simulink model "model_PWM_dspic"  (Simulink 7.4)
settings: Solver=FixedStepDiscrete  StartTime=0.0  StopTime=0.08  FixedStep=0.00001  RelTol=1e-3
undefined symbols (not defined in the file or in its folder): DiscIntNeverNeededParam
libraries: dsPICdrivers x7
settings Model: Creator=ELMAY  LastModifiedBy=ELMAY
settings OptimizationCC: OptimizeModelRefInitCode=on  LifeSpan=1
settings HardwareCC: ProdBitPerInt=16  ProdEndianess=LittleEndian  ProdWordSize=16  ProdHWDeviceType=16-bit Generic
settings RTWCC: SystemTargetFile=dspic.tlc  MakeCommand=make_CreateMPLAB  TemplateMakefile=dspic_pic30_gcc.tmf  PostCodeGenCommand=dsPIC_Compile()  Description=Embedded Target for Microchip dsPIC (real-time)  GenerateReport=on  ProcessScript=dspic_make_rtw_hook  IncludeHyperlinkInReport=on  LaunchReport=on
settings CodeAppCC: IgnoreCustomStorageClasses=off
settings STFCustomTargetCC: IncludeMdlTerminateFcn=off  CombineOutputUpdateFcns=on  SuppressErrorStatus=on  ERTCustomFileBanners=on  SupportContinuousTime=off  SupportNonInlinedSFcns=off  SystemTargetFile=dspic.tlc
settings ERTTargetCC: MultiwordLength=2048  ParMdlRefBuildCompliant=off  CompOptLevelCompliant=off  IncludeMdlTerminateFcn=off  SuppressErrorStatus=on  ERTFirstTimeCompliant=off  ModelStepFunctionPrototypeControlCompliant=off  CPPClassGenCompliant=off  ExtModeMexFile=ext_serial_win32_comm  InlinedParameterPlacement=NonHierarchical  ERTSrcFileBannerTemplate=dsPIC_code_template.cgt  ERTHdrFileBannerTemplate=dsPIC_code_template.cgt  ERTDataSrcFileTemplate=dsPIC_code_template.cgt  ERTDataHdrFileTemplate=dsPIC_code_template.cgt  ERTCustomFileTemplate=dsPIC_main.tlc  ConvertIfToSwitch=off
settings CustomProperty: DataType=string  Value=D:\PROGRA~1\MATLAB\R2009b\bin\win32\gmake

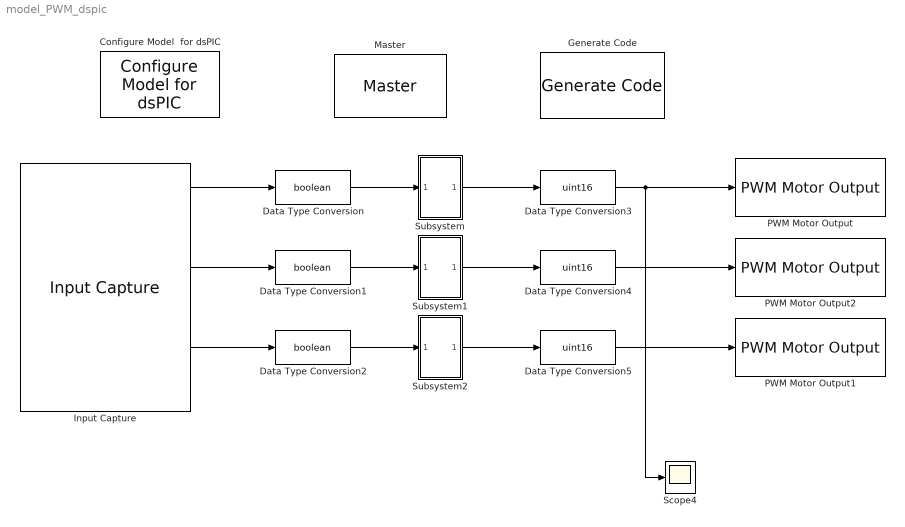
== system model_PWM_dspic ==
  Configure Model  for dsPIC : dsPICdrivers/Simulink Configuration/Configure Model  for dsPIC
  Data Type Conversion : DataTypeConversion  OutDataTypeMode=boolean  OutDataType=sfix(16)  OutScaling=2^0  OutDataTypeStr=boolean
  Data Type Conversion1 : DataTypeConversion  OutDataTypeMode=boolean  OutDataType=sfix(16)  OutScaling=2^0  OutDataTypeStr=boolean
  Data Type Conversion2 : DataTypeConversion  OutDataTypeMode=boolean  OutDataType=sfix(16)  OutScaling=2^0  OutDataTypeStr=boolean
  Data Type Conversion3 : DataTypeConversion  OutDataTypeMode=uint16  OutDataType=sfix(16)  OutScaling=2^0  OutDataTypeStr=uint16
  Data Type Conversion4 : DataTypeConversion  OutDataTypeMode=uint16  OutDataType=sfix(16)  OutScaling=2^0  OutDataTypeStr=uint16
  Data Type Conversion5 : DataTypeConversion  OutDataTypeMode=uint16  OutDataType=sfix(16)  OutScaling=2^0  OutDataTypeStr=uint16
  Generate Code : dsPICdrivers/Simulink Configuration/Generate Code
  Input Capture : dsPICdrivers/Peripheral I//O/Input Capture  Tag=dsPIC_PWM_IC  Priority=5  IntPriority=7  Channel="[ 1 2  7]"  Channel_UP_Down_Periode="[5  5  5]"  MaxChannel="[0.01        0.01        0.01]"  SafeMarge="[10  10  10]"  MaxName=' IC1max , IC2max , IC7max '  Precision="[13.8725      13.8725      13.8725]"  Timer="[2  2  2]"  ChangeDetected="[0  0  0]"  ChangeDetectedPortRef=3  SampleTime=-1  Status=OK
  Master : dsPICdrivers/Master  Tag=dsPIC_MASTER  Priority=1  TimeStepType=Timer1  picType=30f4011  fcy=12e6  Quartz_33f=5e6  PLLActive_33f=off  fcyDesired_33f=0  tmr1="[1  119  1.1842e-014]"  tmr1Info="Time Step : 1e-005  ;   Error : 1.1842e-014%  PR1=119"  tmr2345="[8  0  0  0]"  tmr2345cfg=[-1 -1 -1 -1]  IOautoConf=on  typePort="[ 0  0  0  0  0  0  0  0  0  0  0  0  0  0  0  0  0  0  0  0  6  6  0  0  0  0  0  0  0  0  0  0  0  0  0  0  0  0  0  0  0  0  0  0  0  0  0  0  6  0  0  0  0  0  0  0  0  0  0  0  0  0  0  0  0  0  0  0  0  0  0  0  0  0  0  0  0  0  0  0  0  0  0  0  0  0  0  0  0  0  0  0  0  0  0  0  0  0  0  0  0  0  0  0  0  0  0  0  0  0  0  0 ]"  TRIS="[ 65535  65535  65535  65535  65535  65535  65535 ]"  ADPCFG=48  MasterBusyPort=None  MasterOverloadPort=None  FOSC=HS  ClockSwitchMonitor=Both disabled  TempProtection_33f=TEMP_ON  FPBOR=PBOR_OFF  PWRT=PWRT_OFF  MCLR=MCLR_DIS  ICD=ICS_PGD1  JTAGEN=JTAGEN_OFF  PowerSave=off  OverrideFcy=off  NewFcy=1e6  PR2345="[65535  65535  65535  65535]"
  PWM Motor Output : dsPICdrivers/Peripheral I//O/PWM Motor Output  Tag=dsPIC_PWM_Motor  Priority=5  PWMref=1  PWM12=1  InputEnableChk=off  InputPeriodeChk=off  Channel=[1 ]  TPeriode=0.02  PrescalerValue=16  PeriodeInteger=15000  MaxName='PWM'  Centered=off  HChannelON=off  Info="Nbr Bits : 14.8727  ||  PWM = 30000  ||  Prescaler = 16"  Delay=0  IntPriority=5  nbrPwmChannelPIC=3  Status=OK  DeadTimePrescaleA=0  DeadTimePrescaleB=0  DeadTimeInfo=Dead Time A = 0  DTPWM1a=Prescaler A  DTPWM1i=Prescaler A  DTPWM2a=Prescaler A  DTPWM2i=Prescaler A  DTPWM3a=Prescaler A  DTPWM3i=Prescaler A  DTPWM4a=Prescaler A  DTPWM4i=Prescaler A  DTCON1=0  DTCON2=0
  PWM Motor Output1 : dsPICdrivers/Peripheral I//O/PWM Motor Output  Tag=dsPIC_PWM_Motor  Priority=5  PWMref=1  PWM12=1  InputEnableChk=off  InputPeriodeChk=off  Channel=[3 ]  TPeriode=0.02  PrescalerValue=16  PeriodeInteger=15000  MaxName='PWM'  Centered=off  HChannelON=off  Info="Nbr Bits : 14.8727  ||  PWM = 30000  ||  Prescaler = 16"  Delay=0  IntPriority=5  nbrPwmChannelPIC=3  Status=OK  DeadTimePrescaleA=0  DeadTimePrescaleB=0  DeadTimeInfo=Dead Time A = 0  DTPWM1a=Prescaler A  DTPWM1i=Prescaler A  DTPWM2a=Prescaler A  DTPWM2i=Prescaler A  DTPWM3a=Prescaler A  DTPWM3i=Prescaler A  DTPWM4a=Prescaler A  DTPWM4i=Prescaler A  DTCON1=0  DTCON2=0
  PWM Motor Output2 : dsPICdrivers/Peripheral I//O/PWM Motor Output  Tag=dsPIC_PWM_Motor  Priority=5  PWMref=1  PWM12=1  InputEnableChk=off  InputPeriodeChk=off  Channel=[2 ]  TPeriode=0.02  PrescalerValue=16  PeriodeInteger=15000  MaxName='PWM'  Centered=off  HChannelON=off  Info="Nbr Bits : 14.8727  ||  PWM = 30000  ||  Prescaler = 16"  Delay=0  IntPriority=5  nbrPwmChannelPIC=3  Status=OK  DeadTimePrescaleA=0  DeadTimePrescaleB=0  DeadTimeInfo=Dead Time A = 0  DTPWM1a=Prescaler A  DTPWM1i=Prescaler A  DTPWM2a=Prescaler A  DTPWM2i=Prescaler A  DTPWM3a=Prescaler A  DTPWM3i=Prescaler A  DTPWM4a=Prescaler A  DTPWM4i=Prescaler A  DTCON1=0  DTCON2=0
  Scope4 : Scope
      settings: YMin=-1  YMax=1  SaveName=ScopeData3
  Subsystem : Subsystem
  Subsystem1 : Subsystem
  Subsystem2 : Subsystem
  wires:
  Data Type Conversion/1 -> Subsystem/1(In1)
  Input Capture/1 -> Data Type Conversion/1
  Data Type Conversion1/1 -> Subsystem1/1(In1)
  Input Capture/3 -> Data Type Conversion1/1
  Subsystem1/1(Out1) -> Data Type Conversion4/1
  Input Capture/5 -> Data Type Conversion2/1
  Subsystem2/1(Out1) -> Data Type Conversion5/1
  Data Type Conversion2/1 -> Subsystem2/1(In1)
  Data Type Conversion3/1 -> PWM Motor Output/1, Scope4/1
  Data Type Conversion4/1 -> PWM Motor Output2/1
  Data Type Conversion5/1 -> PWM Motor Output1/1
  Subsystem/1(Out1) -> Data Type Conversion3/1

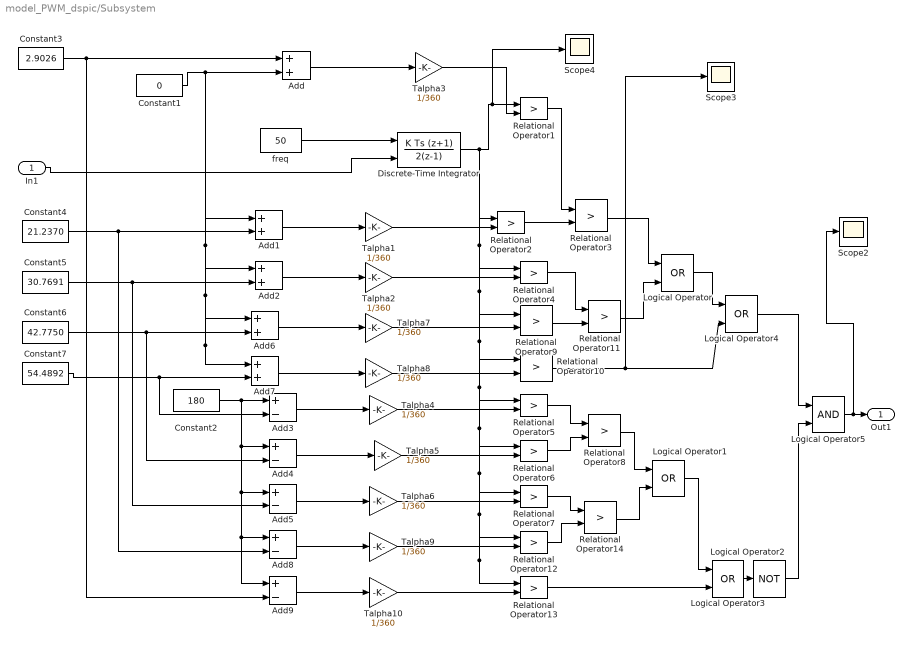
== system model_PWM_dspic/Subsystem ==
  In1 : Inport  OutDataType=fixdt(1, 16)  OutScaling=2^0
  Add{,1..2,6..7} (5 alike) : Sum  OutDataType=fixdt(1, 16)  OutScaling=2^-10
  Add{3..5,8..9} (5 alike) : Sum  Inputs=+-  OutDataType=fixdt(1, 16)  OutScaling=2^-10
  Constant1 : Constant  Value=0  OutDataType=fixdt(1, 16)  OutScaling=2^0
  Constant2 : Constant  Value=180  OutDataType=fixdt(1, 16)  OutScaling=2^0
  Constant3 : Constant  Value=2.9026  OutDataType=fixdt(1, 16)  OutScaling=2^0
  Constant4 : Constant  Value=21.2370  OutDataType=fixdt(1, 16)  OutScaling=2^0
  Constant5 : Constant  Value=30.7691  OutDataType=fixdt(1, 16)  OutScaling=2^0
  Constant6 : Constant  Value=42.7750  OutDataType=fixdt(1, 16)  OutScaling=2^0
  Constant7 : Constant  Value=54.4892  OutDataType=fixdt(1, 16)  OutScaling=2^0
  Discrete-Time Integrator : DiscreteIntegrator  IntegratorMethod=Integration: Trapezoidal  ExternalReset=rising  InitialConditionMode=State only (most efficient)  SampleTime=-1  OutDataType=sfix(16)  OutScaling=2^0  ICPrevOutput=DiscIntNeverNeededParam  ICPrevScaledInput=DiscIntNeverNeededParam
  Logical Operator{,1,3..4} (4 alike) : Logic  Operator=OR  AllPortsSameDT=off  OutDataTypeMode=boolean  LogicDataType=fixdt(0, 8)  OutDataTypeStr=boolean
  Logical Operator2 : Logic  Operator=NOT  AllPortsSameDT=off  OutDataTypeMode=boolean  LogicDataType=fixdt(0, 8)  OutDataTypeStr=boolean
  Logical Operator5 : Logic  AllPortsSameDT=off  OutDataTypeMode=boolean  LogicDataType=fixdt(0, 8)  OutDataTypeStr=boolean
  Relational Operator{1..14} (14 alike) : RelationalOperator  Operator=>  InputSameDT=on
  Scope2 : Scope
  Scope3 : Scope
  Scope4 : Scope
      settings: SaveName=ScopeData2
  Talpha{1..10} (10 alike) : Gain  Gain=1/360  ParameterDataType=sfix(16)  ParameterScaling=2^0  OutDataType=sfix(16)  OutScaling=2^0  SaturateOnIntegerOverflow=on  OutDataTypeStr=Inherit: Same as input  ParamDataTypeStr=Inherit: Same as input
  freq : Constant  Value=50  OutDataType=sfix(16)  OutScaling=2^0
  Out1 : Outport
  wires:
  Add9/1 -> Talpha10/1
  Talpha10/1 -> Relational Operator13/2
  Relational Operator13/1 -> Logical Operator3/2
  Logical Operator2/1 -> Logical Operator5/2
  Logical Operator4/1 -> Logical Operator5/1
  Logical Operator3/1 -> Logical Operator2/1
  Logical Operator1/1 -> Logical Operator3/1
  Relational Operator14/1 -> Logical Operator1/2
  Relational Operator7/1 -> Relational Operator14/1
  Relational Operator12/1 -> Relational Operator14/2
  Talpha9/1 -> Relational Operator12/2
  Add8/1 -> Talpha9/1
  Relational Operator10/1 -> Logical Operator4/2, Scope3/1
  Relational Operator11/1 -> Logical Operator/2
  Relational Operator9/1 -> Relational Operator11/2
  Talpha8/1 -> Relational Operator10/2
  Talpha7/1 -> Relational Operator9/2
  Add7/1 -> Talpha8/1
  Add6/1 -> Talpha7/1
  Constant7/1 -> Add7/2, Add3/2
  Constant6/1 -> Add6/2, Add4/2
  Constant2/1 -> Add3/1, Add4/1, Add5/1, Add8/1, Add9/1
  Add4/1 -> Talpha5/1
  Add5/1 -> Talpha6/1
  Constant5/1 -> Add2/2, Add5/2
  Constant4/1 -> Add1/2, Add8/2
  Add1/1 -> Talpha1/1
  Constant1/1 -> Add/2, Add1/1, Add2/1, Add6/1, Add7/1
  Constant3/1 -> Add/1, Add9/2
  Add/1 -> Talpha3/1
  Relational Operator8/1 -> Logical Operator1/1
  Relational Operator6/1 -> Relational Operator8/2
  Relational Operator5/1 -> Relational Operator8/1
  Talpha6/1 -> Relational Operator7/2
  Talpha5/1 -> Relational Operator6/2
  Add3/1 -> Talpha4/1
  Talpha4/1 -> Relational Operator5/2
  Relational Operator2/1 -> Relational Operator3/2
  Relational Operator3/1 -> Logical Operator/1
  Logical Operator/1 -> Logical Operator4/1
  Relational Operator4/1 -> Relational Operator11/1
  Add2/1 -> Talpha2/1
  Talpha2/1 -> Relational Operator4/2
  Talpha1/1 -> Relational Operator2/2
  freq/1 -> Discrete-Time Integrator/1
  Talpha3/1 -> Relational Operator1/2
  Discrete-Time Integrator/1 -> Relational Operator2/1, Relational Operator4/1, Relational Operator9/1, Relational Operator5/1, Relational Operator6/1, Relational Operator7/1, Relational Operator12/1, Relational Operator13/1, Relational Operator10/1, Relational Operator1/1, Scope4/1
  Relational Operator1/1 -> Relational Operator3/1
  Logical Operator5/1 -> Out1/1, Scope2/1
  In1/1 -> Discrete-Time Integrator/2

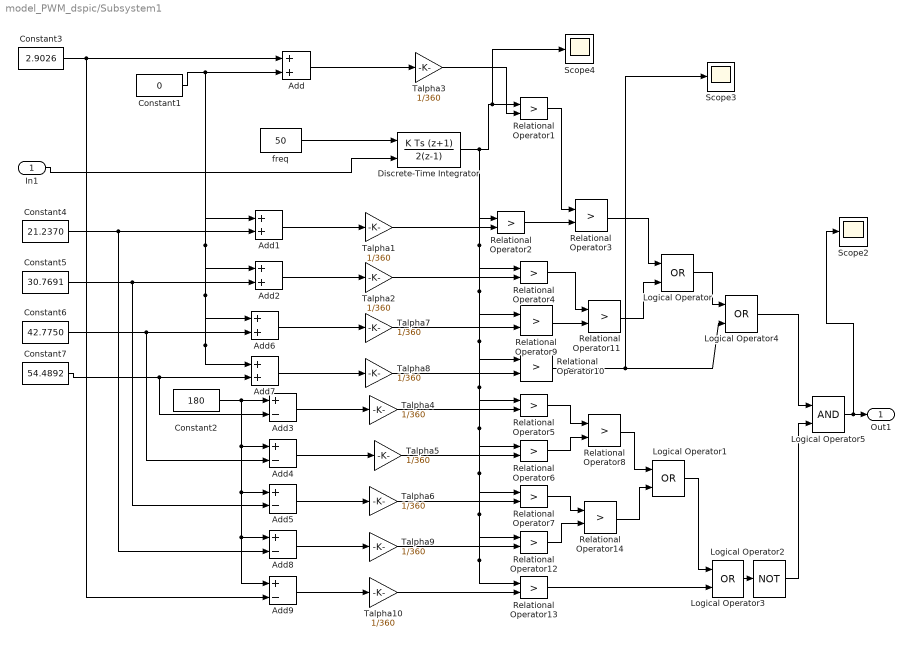
== system model_PWM_dspic/Subsystem1 ==
  In1 : Inport  OutDataType=fixdt(1, 16)  OutScaling=2^0
  Add{,1..2,6..7} (5 alike) : Sum  OutDataType=fixdt(1, 16)  OutScaling=2^-10
  Add{3..5,8..9} (5 alike) : Sum  Inputs=+-  OutDataType=fixdt(1, 16)  OutScaling=2^-10
  Constant1 : Constant  Value=0  OutDataType=fixdt(1, 16)  OutScaling=2^0
  Constant2 : Constant  Value=180  OutDataType=fixdt(1, 16)  OutScaling=2^0
  Constant3 : Constant  Value=2.9026  OutDataType=fixdt(1, 16)  OutScaling=2^0
  Constant4 : Constant  Value=21.2370  OutDataType=fixdt(1, 16)  OutScaling=2^0
  Constant5 : Constant  Value=30.7691  OutDataType=fixdt(1, 16)  OutScaling=2^0
  Constant6 : Constant  Value=42.7750  OutDataType=fixdt(1, 16)  OutScaling=2^0
  Constant7 : Constant  Value=54.4892  OutDataType=fixdt(1, 16)  OutScaling=2^0
  Discrete-Time Integrator : DiscreteIntegrator  IntegratorMethod=Integration: Trapezoidal  ExternalReset=rising  InitialConditionMode=State only (most efficient)  SampleTime=-1  OutDataType=sfix(16)  OutScaling=2^0  ICPrevOutput=DiscIntNeverNeededParam  ICPrevScaledInput=DiscIntNeverNeededParam
  Logical Operator{,1,3..4} (4 alike) : Logic  Operator=OR  AllPortsSameDT=off  OutDataTypeMode=boolean  LogicDataType=fixdt(0, 8)  OutDataTypeStr=boolean
  Logical Operator2 : Logic  Operator=NOT  AllPortsSameDT=off  OutDataTypeMode=boolean  LogicDataType=fixdt(0, 8)  OutDataTypeStr=boolean
  Logical Operator5 : Logic  AllPortsSameDT=off  OutDataTypeMode=boolean  LogicDataType=fixdt(0, 8)  OutDataTypeStr=boolean
  Relational Operator{1..14} (14 alike) : RelationalOperator  Operator=>  InputSameDT=on
  Scope2 : Scope
  Scope3 : Scope
  Scope4 : Scope
      settings: SaveName=ScopeData2
  Talpha{1..10} (10 alike) : Gain  Gain=1/360  ParameterDataType=sfix(16)  ParameterScaling=2^0  OutDataType=sfix(16)  OutScaling=2^0  SaturateOnIntegerOverflow=on  OutDataTypeStr=Inherit: Same as input  ParamDataTypeStr=Inherit: Same as input
  freq : Constant  Value=50  OutDataType=sfix(16)  OutScaling=2^0
  Out1 : Outport
  wires:
  Add9/1 -> Talpha10/1
  Talpha10/1 -> Relational Operator13/2
  Relational Operator13/1 -> Logical Operator3/2
  Logical Operator2/1 -> Logical Operator5/2
  Logical Operator4/1 -> Logical Operator5/1
  Logical Operator3/1 -> Logical Operator2/1
  Logical Operator1/1 -> Logical Operator3/1
  Relational Operator14/1 -> Logical Operator1/2
  Relational Operator7/1 -> Relational Operator14/1
  Relational Operator12/1 -> Relational Operator14/2
  Talpha9/1 -> Relational Operator12/2
  Add8/1 -> Talpha9/1
  Relational Operator10/1 -> Logical Operator4/2, Scope3/1
  Relational Operator11/1 -> Logical Operator/2
  Relational Operator9/1 -> Relational Operator11/2
  Talpha8/1 -> Relational Operator10/2
  Talpha7/1 -> Relational Operator9/2
  Add7/1 -> Talpha8/1
  Add6/1 -> Talpha7/1
  Constant7/1 -> Add7/2, Add3/2
  Constant6/1 -> Add6/2, Add4/2
  Constant2/1 -> Add3/1, Add4/1, Add5/1, Add8/1, Add9/1
  Add4/1 -> Talpha5/1
  Add5/1 -> Talpha6/1
  Constant5/1 -> Add2/2, Add5/2
  Constant4/1 -> Add1/2, Add8/2
  Add1/1 -> Talpha1/1
  Constant1/1 -> Add/2, Add1/1, Add2/1, Add6/1, Add7/1
  Constant3/1 -> Add/1, Add9/2
  Add/1 -> Talpha3/1
  Relational Operator8/1 -> Logical Operator1/1
  Relational Operator6/1 -> Relational Operator8/2
  Relational Operator5/1 -> Relational Operator8/1
  Talpha6/1 -> Relational Operator7/2
  Talpha5/1 -> Relational Operator6/2
  Add3/1 -> Talpha4/1
  Talpha4/1 -> Relational Operator5/2
  Relational Operator2/1 -> Relational Operator3/2
  Relational Operator3/1 -> Logical Operator/1
  Logical Operator/1 -> Logical Operator4/1
  Relational Operator4/1 -> Relational Operator11/1
  Add2/1 -> Talpha2/1
  Talpha2/1 -> Relational Operator4/2
  Talpha1/1 -> Relational Operator2/2
  freq/1 -> Discrete-Time Integrator/1
  Talpha3/1 -> Relational Operator1/2
  Discrete-Time Integrator/1 -> Relational Operator2/1, Relational Operator4/1, Relational Operator9/1, Relational Operator5/1, Relational Operator6/1, Relational Operator7/1, Relational Operator12/1, Relational Operator13/1, Relational Operator10/1, Relational Operator1/1, Scope4/1
  Relational Operator1/1 -> Relational Operator3/1
  Logical Operator5/1 -> Out1/1, Scope2/1
  In1/1 -> Discrete-Time Integrator/2

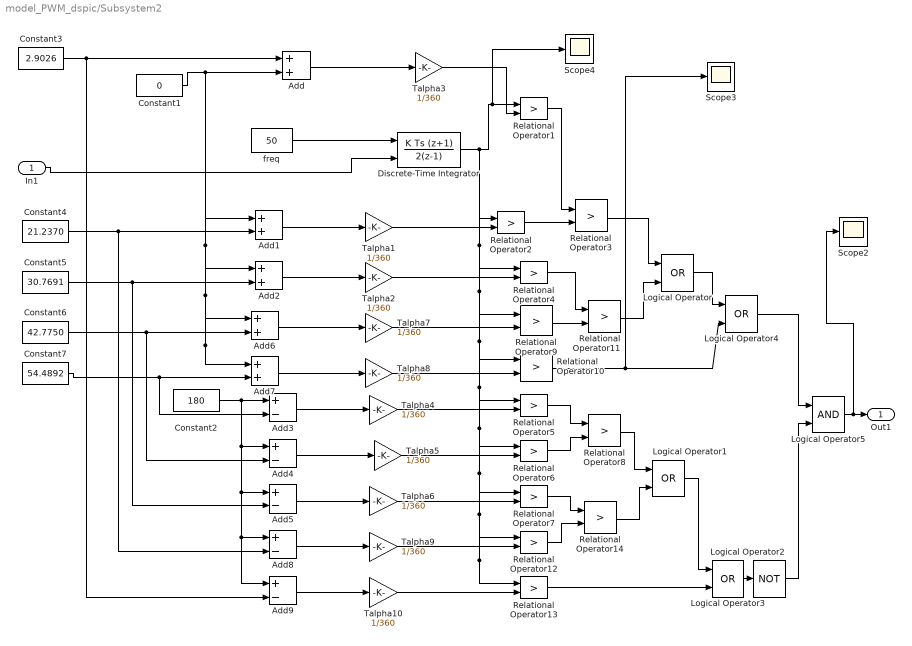
== system model_PWM_dspic/Subsystem2 ==
  In1 : Inport  OutDataType=fixdt(1, 16)  OutScaling=2^0
  Add{,1..2,6..7} (5 alike) : Sum  OutDataType=fixdt(1, 16)  OutScaling=2^-10
  Add{3..5,8..9} (5 alike) : Sum  Inputs=+-  OutDataType=fixdt(1, 16)  OutScaling=2^-10
  Constant1 : Constant  Value=0  OutDataType=fixdt(1, 16)  OutScaling=2^0
  Constant2 : Constant  Value=180  OutDataType=fixdt(1, 16)  OutScaling=2^0
  Constant3 : Constant  Value=2.9026  OutDataType=fixdt(1, 16)  OutScaling=2^0
  Constant4 : Constant  Value=21.2370  OutDataType=fixdt(1, 16)  OutScaling=2^0
  Constant5 : Constant  Value=30.7691  OutDataType=fixdt(1, 16)  OutScaling=2^0
  Constant6 : Constant  Value=42.7750  OutDataType=fixdt(1, 16)  OutScaling=2^0
  Constant7 : Constant  Value=54.4892  OutDataType=fixdt(1, 16)  OutScaling=2^0
  Discrete-Time Integrator : DiscreteIntegrator  IntegratorMethod=Integration: Trapezoidal  ExternalReset=rising  InitialConditionMode=State only (most efficient)  SampleTime=-1  OutDataType=sfix(16)  OutScaling=2^0  ICPrevOutput=DiscIntNeverNeededParam  ICPrevScaledInput=DiscIntNeverNeededParam
  Logical Operator{,1,3..4} (4 alike) : Logic  Operator=OR  AllPortsSameDT=off  OutDataTypeMode=boolean  LogicDataType=fixdt(0, 8)  OutDataTypeStr=boolean
  Logical Operator2 : Logic  Operator=NOT  AllPortsSameDT=off  OutDataTypeMode=boolean  LogicDataType=fixdt(0, 8)  OutDataTypeStr=boolean
  Logical Operator5 : Logic  AllPortsSameDT=off  OutDataTypeMode=boolean  LogicDataType=fixdt(0, 8)  OutDataTypeStr=boolean
  Relational Operator{1..14} (14 alike) : RelationalOperator  Operator=>  InputSameDT=on
  Scope2 : Scope
  Scope3 : Scope
  Scope4 : Scope
      settings: SaveName=ScopeData2
  Talpha{1..10} (10 alike) : Gain  Gain=1/360  ParameterDataType=sfix(16)  ParameterScaling=2^0  OutDataType=sfix(16)  OutScaling=2^0  SaturateOnIntegerOverflow=on  OutDataTypeStr=Inherit: Same as input  ParamDataTypeStr=Inherit: Same as input
  freq : Constant  Value=50  OutDataType=sfix(16)  OutScaling=2^0
  Out1 : Outport
  wires:
  Add9/1 -> Talpha10/1
  Talpha10/1 -> Relational Operator13/2
  Relational Operator13/1 -> Logical Operator3/2
  Logical Operator2/1 -> Logical Operator5/2
  Logical Operator4/1 -> Logical Operator5/1
  Logical Operator3/1 -> Logical Operator2/1
  Logical Operator1/1 -> Logical Operator3/1
  Relational Operator14/1 -> Logical Operator1/2
  Relational Operator7/1 -> Relational Operator14/1
  Relational Operator12/1 -> Relational Operator14/2
  Talpha9/1 -> Relational Operator12/2
  Add8/1 -> Talpha9/1
  Relational Operator10/1 -> Logical Operator4/2, Scope3/1
  Relational Operator11/1 -> Logical Operator/2
  Relational Operator9/1 -> Relational Operator11/2
  Talpha8/1 -> Relational Operator10/2
  Talpha7/1 -> Relational Operator9/2
  Add7/1 -> Talpha8/1
  Add6/1 -> Talpha7/1
  Constant7/1 -> Add7/2, Add3/2
  Constant6/1 -> Add6/2, Add4/2
  Constant2/1 -> Add3/1, Add4/1, Add5/1, Add8/1, Add9/1
  Add4/1 -> Talpha5/1
  Add5/1 -> Talpha6/1
  Constant5/1 -> Add2/2, Add5/2
  Constant4/1 -> Add1/2, Add8/2
  Add1/1 -> Talpha1/1
  Constant1/1 -> Add/2, Add1/1, Add2/1, Add6/1, Add7/1
  Constant3/1 -> Add/1, Add9/2
  Add/1 -> Talpha3/1
  Relational Operator8/1 -> Logical Operator1/1
  Relational Operator6/1 -> Relational Operator8/2
  Relational Operator5/1 -> Relational Operator8/1
  Talpha6/1 -> Relational Operator7/2
  Talpha5/1 -> Relational Operator6/2
  Add3/1 -> Talpha4/1
  Talpha4/1 -> Relational Operator5/2
  Relational Operator2/1 -> Relational Operator3/2
  Relational Operator3/1 -> Logical Operator/1
  Logical Operator/1 -> Logical Operator4/1
  Relational Operator4/1 -> Relational Operator11/1
  Add2/1 -> Talpha2/1
  Talpha2/1 -> Relational Operator4/2
  Talpha1/1 -> Relational Operator2/2
  freq/1 -> Discrete-Time Integrator/1
  Talpha3/1 -> Relational Operator1/2
  Discrete-Time Integrator/1 -> Relational Operator2/1, Relational Operator4/1, Relational Operator9/1, Relational Operator5/1, Relational Operator6/1, Relational Operator7/1, Relational Operator12/1, Relational Operator13/1, Relational Operator10/1, Relational Operator1/1, Scope4/1
  Relational Operator1/1 -> Relational Operator3/1
  Logical Operator5/1 -> Out1/1, Scope2/1
  In1/1 -> Discrete-Time Integrator/2
